simulink model "depthsemantic2"  (R2026b)
settings: Solver=VariableStepAuto
undefined symbols (not defined in the file): Sim3dSensor
libraries: simulink x1, sim3dcameralib x1, sim3dlib x1, uavsim3dlib x1
settings Model: Creator=Shobhit  LastModifiedBy=Shobhit

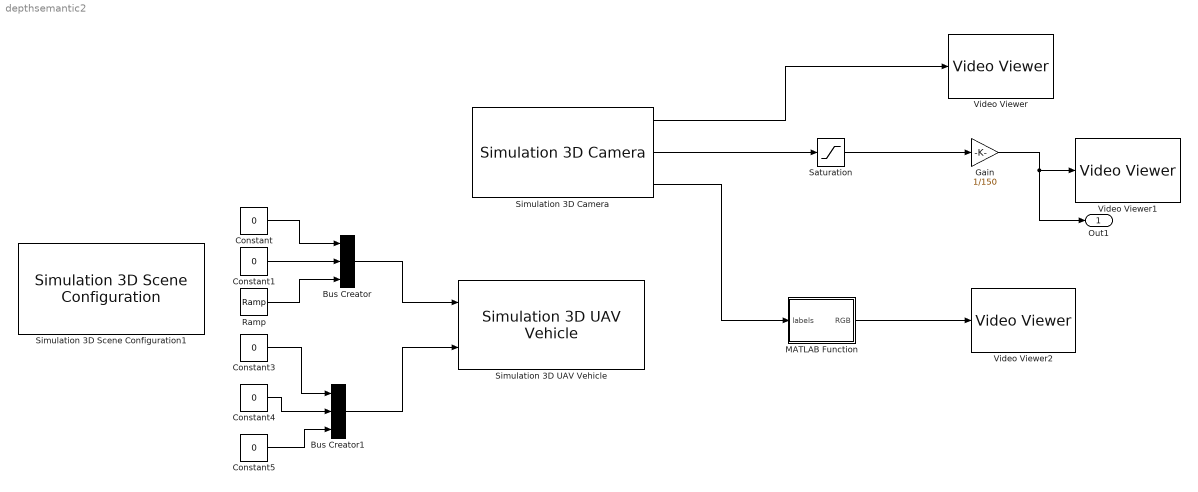
== system depthsemantic2 ==
  Bus Creator : BusCreator  Inputs=3
  Bus Creator1 : BusCreator  Inputs=3
  Constant{,1,3..5} (5 alike) : Constant  Value=0
  Gain : Gain  Gain=1/150
  MATLAB Function : MATLAB Function  TreatAsAtomicUnit=on
  Ramp : simulink/Sources/Ramp  slope=1  start=0  InitialOutput=0
  Saturation : Saturate  UpperLimit=150  LowerLimit=0
  Simulation 3D Camera : sim3dcameralib/Simulation 3D Camera  Priority=1  sensorTag=Sim3dSensor�  sensorId=3  sensorName=Sim3dSensor�  vehTagList={'Custom ...';'Scene Origin';'SimulinkVehicle1';'SimulinkVehicle2'}  vehTag=SimulinkVehicle2  CoordinateSystem=Default  mountLoc=Origin  offsetFlag=off  tmountOffset=[0, 0, 0]  extTmount=off  rmountOffset=[0, 0, 0]  extRmount=off  FocalLength=[1109, 1109]  OpticalCenter=[640, 360]  ImageSize=[720, 1280]  RadialDistortion=[0, 0]  TangentialDistortion=[0, 0]  SensorSkew=0  VisualizeFieldOfView=off  FieldOfViewRange=61  DepthOutportEnabled=on  SemanticOutportEnabled=on  TransformOutportEnabled=off  SampleTime=-1  mountPoint=[0 0 0]  mountOrientation=[0 0 0]  aMode=5  ID=3
      settings: LibrarySourceBlock=sl3dlib/Simulation 3D/Sensors/Simulation 3D Camera
  Simulation 3D Scene Configuration1 : sim3dlib/Simulation 3D Scene Configuration  Priority=0  EnableWindow=on  ViewerType=Default Viewer  ProjectFormat=Default Scenes  SceneDesc=US city block  ProjectName=C:\Program Files\MATLAB\R2026b\toolbox\shared\sim3d_projects\automotive_project_windows\UE\WindowsNoEditor\VehicleSimulation.exe  ScenePath=/Game/Maps/USCityBlock  EnableOpenDRIVE=off  vehTagList={'Custom';'Scene Origin';'SimulinkVehicle2'}  vehTag=SimulinkVehicle2  AttachedCameraRelativeTranslation=[0 0 0]  FreeCameraDefaultInitialTranslation=[-6, 0, 2]  AttachedCameraRelativeRotation=[0, -15, 0]  FreeCameraDefaultInitialRotation=[0, -15, 0]  ViewpointName=Custom  FreeCameraInitialTranslation=[0, 0, 0]  FreeCameraInitialRotation=[0, 0, 0]  OpVisEn=off  Ts=1/60  EnableRemoteAccess=off  SimulationMode=CoSimulation  SimulateUsing=Interpreted execution  EnableAnimationRecording=off  OverrideDefaultRecording=off  AnimationRecordingFileName=sim3dAnimation.mat  AnimationRecordingInterval=[0 inf]  EnableWeather=off  SunAzimuth=90  SunAltitude=40.0  EnableGeospatialSun=off  Latitude=0  Longitude=0  Date=2023-01-01  Time=10:30:00  GeoTimeZone=-5.0  SunDaylightSaving=off  wind=1  clouds=10  EnableVolumetricClouds=off  CloudCoverage=0  CloudAltitude=6  fog=0  rain=0  RaindropsEffect=off  SnowDensity=0  EnableGeospatial=off  TilesetSource=Earth terrain  UseTrueOrigin=off  OriginHeight=200  OriginLatitude=40.744652  OriginLongitude=-73.988864  MapStyle=Aerial  AdditionalAssetIDs=[]  UseAdvancedSunSky=off  SolarTime=11  TimeZone=-5  Day=21  Month=9  Year=2022  UseDaylightSavingTime=on  DSTStartDay=10  DSTStartMonth=3  DSTEndDay=3  DSTEndMonth=11  DSTSwitchHour=2  sensorTag=MainCamera3  sensorId=3  sensorName=MainCamera3  mountLoc=Origin  offsetFlag=off  tmountOffset=[0, 0, 0]  rmountOffset=[0, 0, 0]  HorizontalResolution=1280  VerticalResolution=720  HorizontalFOV=60  mountPoint=[0 0 0]  mountOrientation=[0 0 0]  aMode=4  ID=3  GeoTrigger=Inactive  ViewNameList={'Custom'}  ViewTranslationList={'[0 0 0]'}  ViewRotationList={'[0 0 0]'}
      settings: LibrarySourceBlock=uavsim3dlib/Simulation 3D Scene Configuration
  Simulation 3D UAV Vehicle : uavsim3dlib/Simulation 3D UAV Vehicle  Priority=-1  Mesh=Quadrotor  MeshPath=/MathWorksUAVContent/UAVs/HexaRotorUAV/HexaRotor.HexaRotor  Color=Black  ActorName=SimulinkVehicle2  UseGlobalFrame=off  InitialTranslation=[0 0 0]  InitialRotation=[0 0 0]  InitialTranslationGlobal=[0 0 0]  InitialGeoOrigin=[0 0 0]  InitialRotationGlobal=[0 0 0]  SampleTime=-1  ActorType=SimulinkVehicle  ID=2  aMode=4  ActorTag=SimulinkVehicle2
  Video Viewer : VideoViewer  FigPos=[2 1389 1278 588]
  Video Viewer1 : VideoViewer  FigPos=[1282 1389 1278 588]
  Video Viewer2 : VideoViewer  FigPos=[1282 693 1278 588]
  Out1 : Outport
  wires:
  Constant/1 -> Bus Creator/1
  Constant1/1 -> Bus Creator/2
  Ramp/1 -> Bus Creator/3
  Bus Creator/1 -> Simulation 3D UAV Vehicle/1
  Constant3/1 -> Bus Creator1/1
  Constant4/1 -> Bus Creator1/2
  Constant5/1 -> Bus Creator1/3
  Bus Creator1/1 -> Simulation 3D UAV Vehicle/2
  Simulation 3D Camera/1 -> Video Viewer/1
  Simulation 3D Camera/2 -> Saturation/1
  Saturation/1 -> Gain/1
  Gain/1 -> Out1/1, Video Viewer1/1
  Simulation 3D Camera/3 -> MATLAB Function/1(labels)
  MATLAB Function/1(RGB) -> Video Viewer2/1

== matlab function depthsemantic2/MATLAB Function ==
  data: labels input; RGB output
function RGB = uavlabel2rgb(labels)

coder.extrinsic('label2rgb');

RGB = zeros(720,1280,3,'uint8');

cmap = zeros(256,3);

cmap(1:31,:) = [
    128 0 0
    0 0 0
    72 0 0
    0 0 0
    192 192 192
    128 0 128
    128 64 128
    64 40 222
    128 128 0
    64 0 128
    0 0 0
    192 128 128
    192 128 128
    192 128 128
    192 128 128
    192 128 128
    192 128 128
    0 0 0
    0 0 0
    192 128 128
    192 128 128
    192 128 128
    0 0 0
    192 128 128
    0 0 0
    192 128 128
    0 0 0
    0 0 0
    0 0 0
    0 0 0
    0 0 0
    ] / 255;

RGB(:,:,:) = label2rgb(labels,cmap);

end
